simulink model "RLC_model_1"  (R2025b)
settings: Solver=VariableStepAuto  StartTime=0.0  StopTime=10.0  RelTol=1e-3
undefined symbols (not defined in the file): C, L, R, W0
settings Model: Creator=11  LastModifiedBy=11

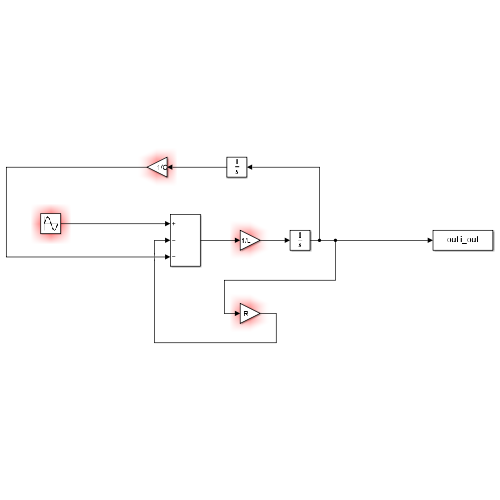
[thumbnail: Simulink's stored preview of the top-level diagram]
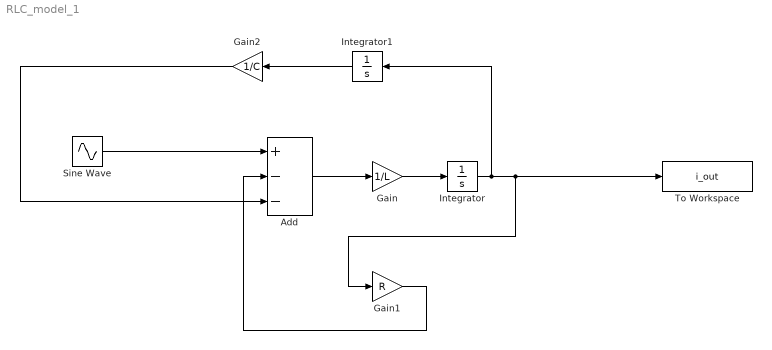
== system RLC_model_1 ==
  Add : Sum  Inputs=+--
  Gain : Gain  Gain=1/L
  Gain1 : Gain  Gain=R
  Gain2 : Gain  Gain=1/C
  Integrator : Integrator
  Integrator1 : Integrator
  Sine Wave : Sin  Frequency=W0  Phase=pi/2  SampleTime=0
  To Workspace : ToWorkspace  VariableName=i_out  SaveFormat=Timeseries  SampleTime=-1
  wires:
  Add/1 -> Gain/1
  Gain/1 -> Integrator/1
  Integrator/1 -> Integrator1/1, Gain1/1, To Workspace/1
  Gain1/1 -> Add/2
  Integrator1/1 -> Gain2/1
  Gain2/1 -> Add/3
  Sine Wave/1 -> Add/1
